simulink model "sf_fixedpoint_iir_filter"  (R2025b)
settings: Solver=FixedStepDiscrete  StartTime=0.0  StopTime=0.1  FixedStep=1/Fs  RelTol=1e-3  EnableMultiTasking=on
PreLoadFcn:
  | Fs = 1000;
  | Fc = 50;
  | [B,A] = butter(1,2*pi*Fc/(Fs/2));
  | b0 = B(1);
  | b1 = B(2);
  | a1 = A(2);
settings Model: Creator=The MathWorks, Inc.  LastModifiedBy=The MathWorks, Inc.
settings SolverCC: AlgebraicLoopSolver=TrustRegion
settings DataIOCC: LimitDataPoints=on  SaveFormat=Array  ReturnWorkspaceOutputs=off
settings OptimizationCC: ReuseModelBlockBuffer=off  ExpressionDepthLimit=2147483647.0  InitFltsAndDblsToZero=on  LifeSpan=inf
settings DebuggingCC: SaveWithParameterizedLinksMsg=none  UnderspecifiedInitializationDetection=Classic  MergeDetectMultiDrivingBlocksExec=none  SignalResolutionControl=TryResolveAllWithWarning  SolverPrmCheckMsg=warning  MultiTaskDSMMsg=warning  MultiTaskCondExecSysMsg=none  ParameterPrecisionLossMsg=none  FcnCallInpInsideContextMsg=warning  UnconnectedInputMsg=warning  UnconnectedOutputMsg=warning  UnconnectedLineMsg=warning  StateNameClashWarn=warning  SFUnexpectedBacktrackingDiag=warning  SFNoUnconditionalDefaultTransitionDiag=warning  SFExecutionAtInitializationDiag=none  ArithmeticOperatorsInVariantConditions=warning
settings HardwareCC: ProdBitPerPointer=32.0  ProdBitPerSizeT=32.0  ProdBitPerPtrDiffT=32.0  ProdLargestAtomicFloat=None  ProdIntDivRoundTo=Undefined  ProdEndianess=Unspecified  ProdWordSize=32.0  ProdHWDeviceType=32-bit Generic
settings ModelReferenceCC: EnableRefExpFcnMdlSchedulingChecks=on  PropagateSignalLabelsOutOfModel=off
settings SFSimCC: SimUseLocalCustomCode=off  SimParseCustomCode=off  CustomCodeUndefinedFunction=UseInterfaceOnly
settings RTWCC: RTWUseLocalCustomCode=off  GPUComputeCapability=3.5
settings CodeAppCC: StateflowObjectComments=on
settings GRTTargetCC: TargetFcnLib=ansi_tfl_tmw.mat  TargetLangStandard=C89/C90 (ANSI)  CombineOutputUpdateFcns=off  GRTInterface=on
settings ConfigComp: CovMetricSettings=dw  CovSaveCumulativeToWorkspaceVar=on  CovSaveSingleToWorkspaceVar=on  CovExternalEMLEnable=off

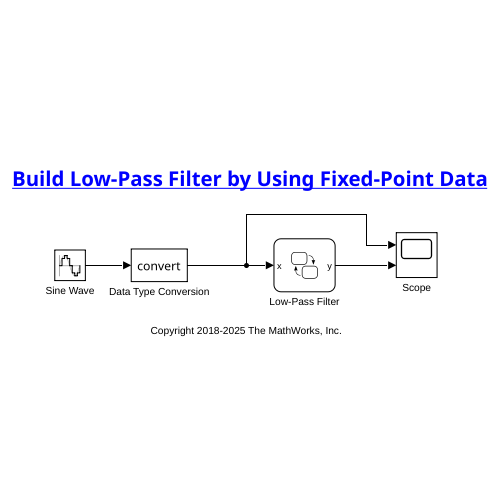
[thumbnail: Simulink's stored preview of the top-level diagram]
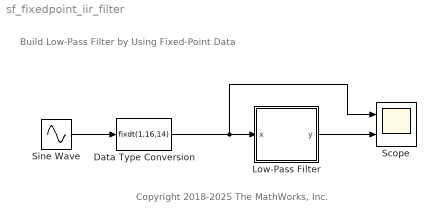
== system sf_fixedpoint_iir_filter ==
  note: Copyright 2018-2025 The MathWorks, Inc.
  note: Build Low-Pass Filter by Using Fixed-Point Data
  Data Type Conversion : DataTypeConversion  OutDataTypeStr=fixdt(1,16,14)  SaturateOnIntegerOverflow=off  RndMeth=Floor
  Low-Pass Filter : Stateflow chart  TreatAsAtomicUnit=on
  Scope : Scope  NumInputPorts=2
      settings: ActiveDisplayYMinimum=-1.24999  ActiveDisplayYMaximum=1.24993
  Sine Wave : Sin  Frequency=2*pi*Fc  SampleTime=1/Fs
  wires:
  Data Type Conversion/1 -> Low-Pass Filter/1(x), Scope/1
  Sine Wave/1 -> Data Type Conversion/1
  Low-Pass Filter/1(y) -> Scope/2

== stateflow chart sf_fixedpoint_iir_filter/Low-Pass Filter ==
  (default) -> (junction 3) : {
      | y = x*b0 + x_n1*b1 - y_n1*a1;
      | x_n1 = x;
      | y_n1 = y;
      | }
  data: x input; b0 parameter fixdt(1,16,15); y_n1 local fixdt(1,16,10); a1 parameter fixdt(1,16,15); y output fixdt(1,16,10); x_n1 local fixdt(1,16,12); b1 parameter fixdt(1,16,15)
